simulink model "sf_power_window"  (R2025b)
settings: Solver=FixedStepAuto  StartTime=0.0  StopTime=inf  FixedStep=0.1  RelTol=1e-3  EnableMultiTasking=on
PreLoadFcn:
  | load sf_power_window_buses;
StopFcn:
  | delete(app)
CloseFcn:
  | clear app
  | clear app_lamps
  | clear app_switches
  | clear servo_commands
settings Model: PacingRate=0.500000  Creator=The MathWorks, Inc.  LastModifiedBy=The MathWorks, Inc.
settings SolverCC: AlgebraicLoopSolver=TrustRegion  MaxZcPerStep=1.0
settings DataIOCC: LimitDataPoints=on  SaveFormat=Array  SaveOutput=off  SaveTime=off  ReturnWorkspaceOutputs=off
settings OptimizationCC: ReuseModelBlockBuffer=off  LifeSpan=inf
settings DebuggingCC: SolverPrmCheckMsg=warning  UnconnectedInputMsg=warning  UnconnectedOutputMsg=warning  UnconnectedLineMsg=warning  AllowSymbolicDim=off  SFUnexpectedBacktrackingDiag=warning  SFNoUnconditionalDefaultTransitionDiag=warning  SFExecutionAtInitializationDiag=none  ArithmeticOperatorsInVariantConditions=warning
settings HardwareCC: ProdBitPerPointer=32.0  ProdBitPerSizeT=32.0  ProdBitPerPtrDiffT=32.0  ProdLargestAtomicFloat=None  ProdIntDivRoundTo=Undefined  ProdEndianess=Unspecified  ProdWordSize=32.0  ProdHWDeviceType=32-bit Generic
settings ModelReferenceCC: EnableRefExpFcnMdlSchedulingChecks=on  PropagateSignalLabelsOutOfModel=off
settings SFSimCC: SimUseLocalCustomCode=off  CustomCodeUndefinedFunction=UseInterfaceOnly
settings RTWCC: RTWUseLocalCustomCode=off  GPUComputeCapability=3.5  DLArmComputeVersion=19.05
settings CodeAppCC: StateflowObjectComments=on
settings GRTTargetCC: TargetLangStandard=C89/C90 (ANSI)
settings ConfigComp: CovMetricSettings=dw  CovSaveCumulativeToWorkspaceVar=on  CovSaveSingleToWorkspaceVar=on  CovExternalEMLEnable=off  CovSFcnEnable=off

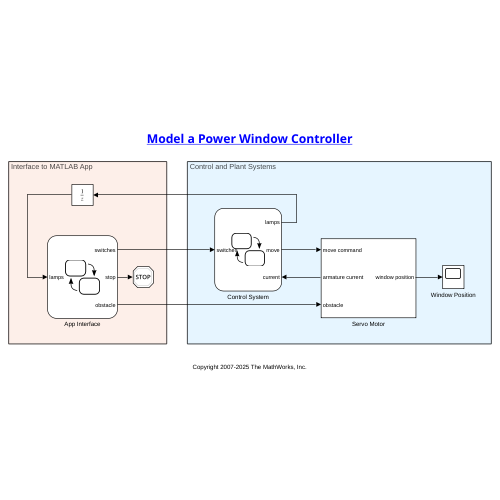
[thumbnail: Simulink's stored preview of the top-level diagram]
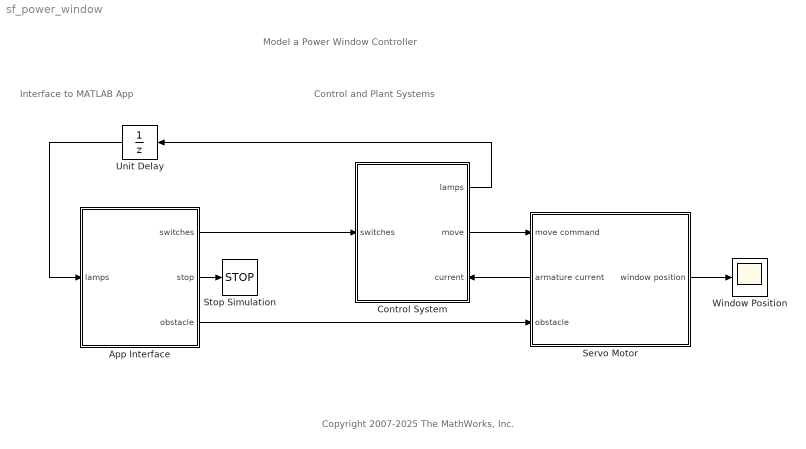
== system sf_power_window ==
  note: Control and Plant Systems
  note: Interface to MATLAB App
  note: Copyright 2007-2025 The MathWorks, Inc.
  note: Model a Power Window Controller
  App Interface : Stateflow chart  TreatAsAtomicUnit=on
      settings: PortSchema="{\"entries\":[{\"content\":{\"sides\":[{\"content\":{\"connectorIds\":[\"In1\"]},\"type\":\"ConnectorPlacement.EquallySpacedRectSide\",\"uuid\":\"e1ad66b1-e568-496f-9e45-7c9e02fee1cc\"},{\"content\":{\"connectorIds\":[\"Out1\",\"Out3\",\"Out2\"],\"side\":\"RIGHT\"},\"type\":\"ConnectorPlacement.EquallySpacedRectSide\",\"uuid\":\"048571b2-7846-48ed-94de-fbaeee814e01\"},{\"content\":{\"connectorIds\":[],\"side\":\"TOP\"},\"type\":\"ConnectorPlacement.EquallySpacedRectSide\",\"uuid\":\"c61124e7-ab7e-45c9-8839-f871c3452aea\"},{\"content\":{\"connectorIds\":[],\"side\":\"HIDDEN\"},\"type\":\"ConnectorPlacement.EquallySpacedRectSide\",\"uuid\":\"2f553fa9-fcee-46d5-a9a9-20753cb5e502\"}]},\"type\":\"ConnectorPlacement.EquallySpacedConnector\",\"uuid\":\"01581893-abfd-4521-bff8-aba671a785a7\"}],\"packageUris\":[\"http://schema.mathworks.com/mf0/Connector/R2020b\"],\"version\":\"1.0\"}"
  Control System : Stateflow chart  TreatAsAtomicUnit=on
      settings: PortSchema="{\"entries\":[{\"content\":{\"sides\":[{\"content\":{\"connectorIds\":[\"In1\"]},\"type\":\"ConnectorPlacement.EquallySpacedRectSide\",\"uuid\":\"956dd6a2-1182-4713-a68f-9bb5f3c20574\"},{\"content\":{\"connectorIds\":[\"Out2\",\"Out1\",\"In2\"],\"side\":\"RIGHT\"},\"type\":\"ConnectorPlacement.EquallySpacedRectSide\",\"uuid\":\"f7d18ef9-efa5-4a0e-963a-79cd1ad1edb5\"},{\"content\":{\"connectorIds\":[],\"side\":\"TOP\"},\"type\":\"ConnectorPlacement.EquallySpacedRectSide\",\"uuid\":\"baea5081-ec8a-4033-b7a7-850772f8ca5b\"},{\"content\":{\"connectorIds\":[],\"side\":\"HIDDEN\"},\"type\":\"ConnectorPlacement.EquallySpacedRectSide\",\"uuid\":\"5aa78869-e583-4ca7-a93f-6bbb3f73db76\"}]},\"type\":\"ConnectorPlacement.EquallySpacedConnector\",\"uuid\":\"dd196b15-55ef-4a17-bf3e-b9b776d3c728\"}],\"packageUris\":[\"http://schema.mathworks.com/mf0/Connector/R2020b\"],\"version\":\"1.0\"}"
  Servo Motor : Subsystem
      settings: PortSchema="{\"entries\":[{\"content\":{\"sides\":[{\"content\":{\"connectorIds\":[\"In1\",\"Out2\",\"In2\"]},\"type\":\"ConnectorPlacement.EquallySpacedRectSide\",\"uuid\":\"b0d36c6e-df2b-4eba-abc8-e692efa24438\"},{\"content\":{\"connectorIds\":[\"Out1\"],\"side\":\"RIGHT\"},\"type\":\"ConnectorPlacement.EquallySpacedRectSide\",\"uuid\":\"c7740b09-28d0-44f6-9d1c-d0fe693b5449\"},{\"content\":{\"connectorIds\":[],\"side\":\"TOP\"},\"type\":\"ConnectorPlacement.EquallySpacedRectSide\",\"uuid\":\"07351fac-2541-4cde-8088-c551794b3695\"},{\"content\":{\"connectorIds\":[],\"side\":\"BOTTOM\"},\"type\":\"ConnectorPlacement.EquallySpacedRectSide\",\"uuid\":\"5e661dee-174a-4e07-a2a1-8f9467db526e\"},{\"content\":{\"connectorIds\":[],\"side\":\"HIDDEN\"},\"type\":\"ConnectorPlacement.EquallySpacedRectSide\",\"uuid\":\"8e3b5e25-b078-4e38-8079-db63e0c14aa7\"}]},\"type\":\"ConnectorPlacement.EquallySpacedConnector\",\"uuid\":\"70c02508-5e69-4de9-84f4-f82bbc88e4ad\"}],\"packageUris\":[\"http://schema.mathworks.com/mf0/Connector/R2020b\"],\"version\":\"1.0\"}"
  Stop Simulation : Stop
  Unit Delay : UnitDelay  SampleTime=-1  HasFrameUpgradeWarning=on
  Window Position : Scope
      settings: ActiveDisplayYMinimum=-0.425  ActiveDisplayYMaximum=3.825
  wires:
  Control System/1(move) -> Servo Motor/1(move command)
  Servo Motor/1(window position) -> Window Position/1
  Servo Motor/2(armature current) -> Control System/2(current)
  App Interface/1(switches) -> Control System/1(switches)
  App Interface/3(stop) -> Stop Simulation/1
  Control System/2(lamps) -> Unit Delay/1
  Unit Delay/1 -> App Interface/1(lamps)
  App Interface/2(obstacle) -> Servo Motor/2(obstacle)

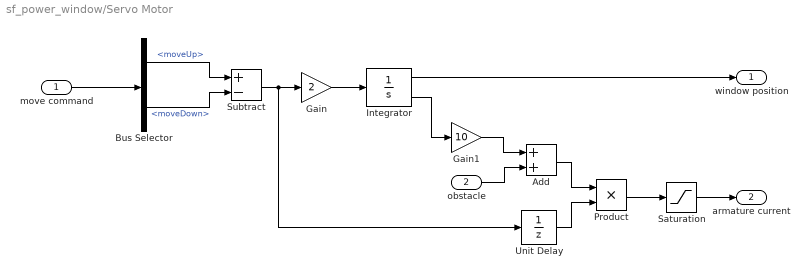
== system sf_power_window/Servo Motor ==
  move command : Inport
  obstacle : Inport  Port=2
  Add : Sum
  Bus Selector : BusSelector  DialogController=Simulink.DDGSource_BusSelector  OutputSignals=moveUp,moveDown
  Gain : Gain  Gain=2
  Gain1 : Gain  Gain=10
  Integrator : Integrator  LimitOutput=on  UpperSaturationLimit=10  LowerSaturationLimit=0  ShowSaturationPort=on
  Product : Product
  Saturation : Saturate  UpperLimit=10  LowerLimit=0
  Subtract : Sum  Inputs=+-  OutDataTypeStr=double
  Unit Delay : UnitDelay  SampleTime=-1  HasFrameUpgradeWarning=on
  window position : Outport
  armature current : Outport  Port=2
  wires:
  Integrator/1 -> window position/1
  Subtract/1 -> Gain/1, Unit Delay/1
  Gain/1 -> Integrator/1
  Unit Delay/1 -> Product/2
  Bus Selector/2 -> Subtract/2  "<moveDown>"
  Bus Selector/1 -> Subtract/1  "<moveUp>"
  move command/1 -> Bus Selector/1
  obstacle/1 -> Add/2
  Integrator/2 -> Gain1/1
  Gain1/1 -> Add/1
  Add/1 -> Product/1
  Saturation/1 -> armature current/1
  Product/1 -> Saturation/1

== stateflow chart sf_power_window/App Interface ==
  state InterfaceFromApp
    en:
    coder.extrinsic('sf_power_window_app','updateLamps');
    app = sf_power_window_app(this);
    initializeData();
    du:
    if hasChanged(lamps)
    updateLamps(app);
    end
    state initializeData [function]
      (default) -> (junction 75) : {
          |  switches.driver_up = false;
          |  switches.driver_down = false;
          |  switches.passenger_up = false;
          |  switches.passenger_down = false;
          |  obstacle = false;
          |  stop = false;
          | }
  (default) -> InterfaceFromApp
  data: switches output Bus: app_switches; obstacle output boolean size=1; stop output boolean size=1; app local; lamps input Bus: app_lamps

== stateflow chart sf_power_window/Control System ==
  state Switch [parallel]
    en:
    initializeLamps();
    du:
    detectObstacles();
    checkSwitches();
    settings: executionOrder=1
    state initializeLamps [function]
      (default) -> (junction 283) : {
          |  lamps.up = false;
          |  lamps.down = false;
          |  lamps.automode = false;
          |  lamps.obstacle = false;
          |  lamps.timeout = false;
          | }
    state detectObstacles [function]
      (default) -> (junction 259)
      (junction 259) -> (junction 262) [order 1] : [current > 1]
      (junction 262) -> (junction 270) : {send(ENDSTOP,Logic);}
      (junction 259) -> (junction 264) [order 2]
      (junction 264) -> (junction 278) [order 1] : [current > 0]
      (junction 278) -> (junction 268) : {send(OBSTACLE,Logic);}
      (junction 264) -> (junction 274) [order 2]
  state go [group]
    state neutral [function]
      (default) -> (junction 165) : {
          |  move.moveUp = false;
          |  move.moveDown = false;
          |  lamps.up = false;
          |  lamps.down = false;
          | }
    state up [function]
      (default) -> (junction 238) : {
          |  move.moveUp = true;
          |  move.moveDown = false;
          |  lamps.up = true;
          |  lamps.down = false;
          | }
    state down [function]
      (default) -> (junction 240) : {
          |  move.moveUp = false;
          |  move.moveDown = true;
          |  lamps.up = false;
          |  lamps.down = true;
          | }
  state Logic [parallel]
    settings: executionOrder=2
    state Stop
      en:
      go.neutral();
      state Mode [parallel]
        settings: executionOrder=1
        state Waiting
        state Ready
          en: lamps.timeout = false;
        (default) -> Waiting
        Waiting -> Ready : NEUTRAL
      state Position [parallel]
        settings: executionOrder=2
        state InTheMiddle
        state NearTop
        state NearBottom
        (default) -> InTheMiddle
        (junction 167) -> NearTop [order 1] : [in(Move.Direction.Up)]
        (junction 167) -> (junction 38) [order 2]
        (junction 38) -> NearBottom
      (junction 170) -> (junction 167)
    state Move
      state Direction [parallel]
        settings: executionOrder=1
        state Down
          en: go.down();
        state Error
        state Up
          en: go.up();
        (default) -> (junction 28)
        (junction 28) -> Down [order 1] : DOWN
        (junction 28) -> (junction 26) [order 2]
        (junction 26) -> Error [order 2]
        (junction 26) -> Up [order 1] : UP
      state Mode [parallel]
        settings: executionOrder=2
        state Initializing
        state Manual
        state Auto
          en: lamps.automode = true;
          ex: lamps.automode = false;
        (default) -> Initializing
        Initializing -> (junction 244) [order 1] : NEUTRAL
        (junction 244) -> Auto : after(.5,sec)
        Initializing -> Manual [order 2] : after(1,sec)
      Down -> Move : UP
      Up -> Move : DOWN
      Auto -> Move : UP || DOWN
    state EmergencyDown
      en:
      lamps.obstacle = true;
      go.down();
      ex:
      lamps.obstacle = false;
    (default) -> Stop
    Move -> Stop [order 1] : after(FAILSAFE_TIMEOUT,sec){lamps.timeout = true;}
    EmergencyDown -> Stop [order 1] : after(1,sec)
    Move -> EmergencyDown [order 2] : OBSTACLE
    EmergencyDown -> (junction 233) [order 2] : ENDSTOP
    (junction 233) -> (junction 170)
    Move -> (junction 233) [order 3] : ENDSTOP
    (junction 95) -> Stop
    Initializing -> (junction 95) [order 3] : NEUTRAL
    (junction 199) -> (junction 95)
    InTheMiddle -> (junction 46) : UP || DOWN
    (junction 46) -> (junction 99)
    Manual -> (junction 199) : NEUTRAL
    NearTop -> (junction 99) : DOWN
    (junction 99) -> (junction 16)
    NearBottom -> (junction 16) : UP
    (junction 16) -> Move : [in(Stop.Mode.Ready)]
  data: move output Bus: servo_commands; FAILSAFE_TIMEOUT constant uint16 size=1 =10; switches input Bus: app_switches size=1; current input; lamps output Bus: app_lamps
  events: NEUTRAL local FUNCTION_CALL_EVENT; UP local FUNCTION_CALL_EVENT; DOWN local FUNCTION_CALL_EVENT; ENDSTOP local RISING_EDGE_EVENT; OBSTACLE local RISING_EDGE_EVENT
  function checkSwitches:
    | function checkSwitches
    | 
    | aVarTruthTableCondition_1 = false;
    | aVarTruthTableCondition_2 = false;
    | aVarTruthTableCondition_3 = false;
    | aVarTruthTableCondition_4 = false;
    | 
    | 
    | 
    | aVarTruthTableCondition_1 = logical(switches.driver_up);
    | 
    | 
    | aVarTruthTableCondition_2 = logical(switches.driver_down);
    | 
    | 
    | aVarTruthTableCondition_3 = logical(switches.passenger_up);
    | 
    | 
    | aVarTruthTableCondition_4 = logical(switches.passenger_down);
    | 
    | if (aVarTruthTableCondition_1 && ~aVarTruthTableCondition_2)
    |     aFcnTruthTableAction_1();
    | elseif (~aVarTruthTableCondition_1 && aVarTruthTableCondition_2)
    |     aFcnTruthTableAction_2();
    | elseif (~aVarTruthTableCondition_1 && ~aVarTruthTableCondition_2 && aVarTruthTableCondition_3 && ~aVarTruthTableCondition_4)
    |     aFcnTruthTableAction_1();
    | elseif (~aVarTruthTableCondition_1 && ~aVarTruthTableCondition_2 && ~aVarTruthTableCondition_3 && aVarTruthTableCondition_4)
    |     aFcnTruthTableAction_2();
    | else % Default
    |     aFcnTruthTableAction_3();
    | end
    | 
    | function aFcnTruthTableAction_1()
    | 
    | % Move Up
    | 
    | send(UP,Logic);
    | 
    | function aFcnTruthTableAction_2()
    | 
    | % Move Down
    | 
    | send(DOWN,Logic);
    | 
    | function aFcnTruthTableAction_3()
    | 
    | % Stay Neutral
    | 
    | send(NEUTRAL,Logic);
